simulink model "SolarTrackerSystem"  (R2026b)
settings: Solver=FixedStepDiscrete  StartTime=0  StopTime=86340  FixedStep=60
model workspace (MAT data in the model file):
  targetInput = timeseries
  targetInput.Name = 'unnamed'
  targetInput.DataInfo = tsdata.datametadata
  targetInput.DataInfo.Interpolation = tsdata.interpolation
  targetInput.DataInfo.Interpolation.Fhandle : function handle (value not decoded)
  targetInput.DataInfo.Interpolation.Name = 'linear'
  targetInput.TimeInfo = tsdata.timemetadata
  targetInput.TimeInfo.Length = 1440
  targetInput.TimeInfo.DuplicateTimes = 0
  targetInput.TimeInfo.Time_ = [0 60 120 180 240 300 360 420 480 540 600 660 ... (1440 elements, 1440x1)]
  targetInput.TimeInfo.Initialized = 1
  targetInput.QualityInfo = tsdata.qualmetadata
  targetInput.Data_ = [0 0 0 0 0 0 0 0 0 0 0 0 ... (4320 elements, 1440x3)]
  weatherInput = timeseries
  weatherInput.Name = 'unnamed'
  weatherInput.DataInfo = tsdata.datametadata
  weatherInput.DataInfo.Interpolation = tsdata.interpolation
  weatherInput.DataInfo.Interpolation.Fhandle : function handle (value not decoded)
  weatherInput.DataInfo.Interpolation.Name = 'linear'
  weatherInput.TimeInfo = tsdata.timemetadata
  weatherInput.TimeInfo.Length = 1440
  weatherInput.TimeInfo.DuplicateTimes = 0
  weatherInput.TimeInfo.Time_ = [0 60 120 180 240 300 360 420 480 540 600 660 ... (1440 elements, 1440x1)]
  weatherInput.TimeInfo.Initialized = 1
  weatherInput.QualityInfo = tsdata.qualmetadata
  weatherInput.Data_ = [0 0 0 0 0 0 0 0 0 0 0 0 ... (10080 elements, 1440x7)]
settings Model: Creator=Ayush  LastModifiedBy=Ayush

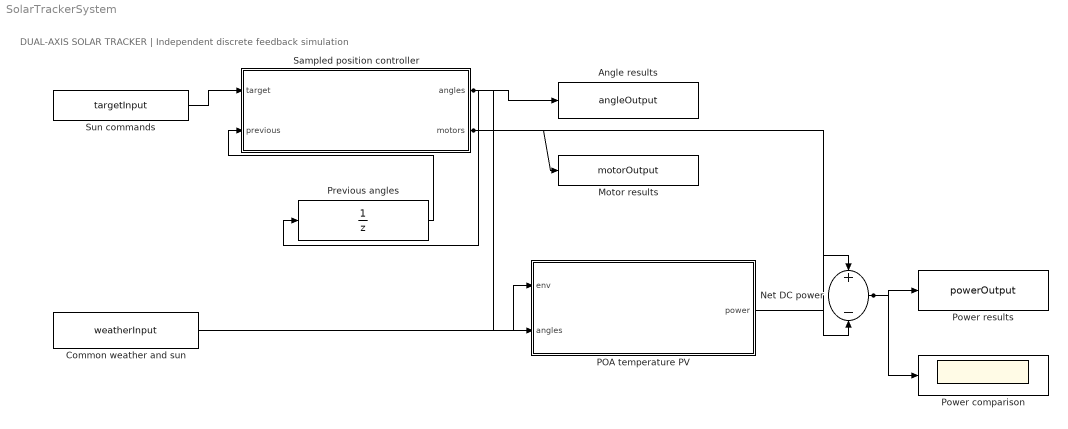
== system SolarTrackerSystem ==
  note: DUAL-AXIS SOLAR TRACKER | Independent discrete feedback simulation
  Angle results : ToWorkspace  VariableName=angleOutput  SaveFormat=Timeseries  SampleTime=-1
  Common weather and sun : FromWorkspace  VariableName=weatherInput  Interpolate=off  OutputAfterFinalValue=Holding final value
  Motor results : ToWorkspace  VariableName=motorOutput  SaveFormat=Timeseries  SampleTime=-1
  Net DC power : Sum  Inputs=+-
  POA temperature PV : MATLAB Function  TreatAsAtomicUnit=on
  Power comparison : Scope
  Power results : ToWorkspace  VariableName=powerOutput  SaveFormat=Timeseries  SampleTime=-1
  Previous angles : UnitDelay  InitialCondition=[0; 180; 90]  SampleTime=60
  Sampled position controller : MATLAB Function  TreatAsAtomicUnit=on
  Sun commands : FromWorkspace  VariableName=targetInput  Interpolate=off  OutputAfterFinalValue=Holding final value
  wires:
  Sun commands/1 -> Sampled position controller/1(target)
  Previous angles/1 -> Sampled position controller/2(previous)
  Sampled position controller/1(angles) -> Previous angles/1, POA temperature PV/2(angles), Angle results/1
  Sampled position controller/2(motors) -> Motor results/1, Net DC power/2
  Common weather and sun/1 -> POA temperature PV/1(env)
  POA temperature PV/1(power) -> Net DC power/1
  Net DC power/1 -> Power results/1, Power comparison/1

== matlab function SolarTrackerSystem/Sampled position controller ==
  data: target input; angles output; previous input; motors output
function [angles,motors]=controller(target,previous)
err=target-previous;
err(abs(err)<=1)=0;
move=max(-12,min(12,err));
angles=previous+move;
motors=[0; 0.05+8*abs(move(1))/12; 0.05+8*(abs(move(2))+abs(move(3)))/12];
end

== matlab function SolarTrackerSystem/POA temperature PV ==
  data: env input; power output; angles input
function power=pv(env,angles)
normal=[0 -0.497796131004339 0.867294074669666; sin(angles(1)*pi/180) 0 cos(angles(1)*pi/180); cos(angles(3)*pi/180)*sin(angles(2)*pi/180) cos(angles(3)*pi/180)*cos(angles(2)*pi/180) sin(angles(3)*pi/180)];
power=zeros(3,1);
for j=1:3
mu=max(0,normal(j,:)*env(5:7));
c=normal(j,3);
poa=env(1)*mu+env(2)*(1+c)/2+0.2*env(3)*(1-c)/2;
temp=env(4)+(45-20)/800*poa;
power(j)=400*poa/1000*max(0,1+-0.004*(temp-25))*(1-0.1);
end
end
